simulink model "BLDC_simscape"  (R2025b)
settings: Solver=ode23t  StartTime=0.0  StopTime=10.0  RelTol=1e-3
undefined symbols (not defined in the file or in its folder): Mosfet_class, PermanentMagnetSynchrono_class
libraries: nesl_utility x26, fl_lib x22, ee_lib x10, simulink x6, eeTransforms x2, elec_conv_HighZElecRef x1, slpidlib x1
(part 2 of 2)

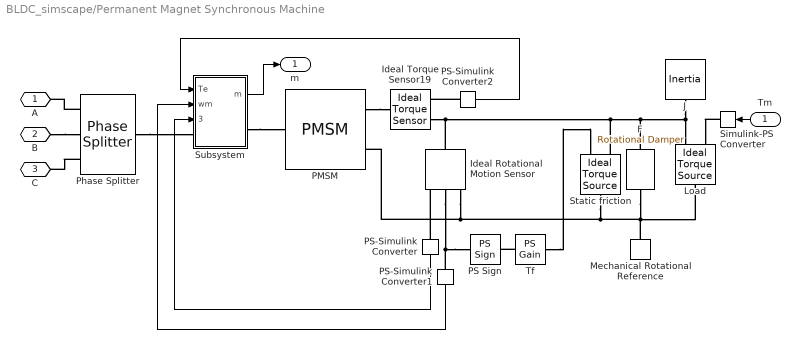
== system BLDC_simscape/Permanent Magnet Synchronous Machine ==
  Tm : Inport
  F : fl_lib/Mechanical/Rotational Elements/Rotational Damper  D=0.0004924 N*m/(rad/s)  w_specify=on  w_priority=High  w=0 rad/s  w_nominal_specify=off  w_nominal_value=1  w_nominal_unit=rad/s  t_specify=off  t_priority=None  t=0 N*m  t_nominal_specify=off  t_nominal_value=1  t_nominal_unit=N*m
  Ideal Rotational Motion Sensor : fl_lib/Mechanical/Mechanical Sensors/Ideal Rotational Motion Sensor  reference=foundation.enum.MeasurementReference.difference  acceleration_port=false  velocity_port=true  position_port=true  wrap_angle=simscape.enum.onoff.off  offset=0 deg
  Ideal Torque Sensor19 : fl_lib/Mechanical/Mechanical Sensors/Ideal Torque Sensor
  J : fl_lib/Mechanical/Rotational Elements/Inertia  inertia=0.0027 kg*m^2  num_ports=foundation.enum.numPorts2.one  w_specify=on  w_priority=High  w=0 rad/s  w_nominal_specify=off  w_nominal_value=1  w_nominal_unit=rad/s  t_specify=off  t_priority=None  t=0 N*m  t_nominal_specify=off  t_nominal_value=1  t_nominal_unit=N*m
  Load : fl_lib/Mechanical/Mechanical Sources/Ideal Torque Source
  Mechanical Rotational Reference : fl_lib/Mechanical/Rotational Elements/Mechanical Rotational Reference
  PMSM : ee_lib/Electromechanical/Permanent Magnet/PMSM  port_option=ee.enum.threePhasePort.composite  winding_type=ee.enum.statorconnection.wye  machine_param=ee.enum.pmsm.parameterization.constant  nPolePairs=4  pmflux_param=1  pm_flux_linkage=PermanentMagnetSynchrono_class('Torque Tm',[0.0027 0.0004924 4 0],4,'Flux linkage established by magnets (V.s)',0.1194,86.6271,0.7164,'90 degrees behind phase A axis (modified Park)',[0 0 0 0],'Sinusoidal',120,'3',[0 0 0 0 0 0]).objParamMappingDerived.NewDerivedParam.pm_flux_linkage Wb  torque_constant=0.18 N*m/A  back_emf_constant=0.18 V/(rad/s)  stator_param=1  Ld=0.000395 H  Lq=0.000395 H  idVec=[-200, 0, 200] A  iqVec=[-200, 0, 200] A  LdMatrix=0.0002 * ones(3, 3) H  LqMatrix=0.0002 * ones(3, 3) H  PmMatrix=0.1 * ones(3, 3) Wb  ktMatrix=0.18 * ones(3, 3) N*m/A  keMatrix=0.18 * ones(3, 3) V/(rad/s)  L0=1e-09 H  Ls=0.0002 H  Lm=-0.00002 H  Ms=0.00002 H  Rs=0.7 Ohm  zero_sequence=0  axes_param=1  loss_param=ee.enum.ironloss.none  losses_oc=[0, 0, 0] W  losses_sc=[0, 0, 0] W  f_losses=60 Hz  Isc_losses=95 A  J=0 kg*m^2  lam=0 N*m/(rad/s)  i_d_specify=on  i_d_priority=High  i_d=PermanentMagnetSynchrono_class('Torque Tm',[0.0027 0.0004924 4 0],4,'Flux linkage established by magnets (V.s)',0.1194,86.6271,0.7164,'90 degrees behind phase A axis (modified Park)',[0 0 0 0],'Sinusoidal',120,'3',[0 0 0 0 0 0]).objParamMappingDerived.NewDerivedParam.i_d A  i_d_nominal_specify=off  i_d_nominal_value=1  i_d_nominal_unit=A  i_q_specify=on  i_q_priority=High  i_q=PermanentMagnetSynchrono_class('Torque Tm',[0.0027 0.0004924 4 0],4,'Flux linkage established by magnets (V.s)',0.1194,86.6271,0.7164,'90 degrees behind phase A axis (modified Park)',[0 0 0 0],'Sinusoidal',120,'3',[0 0 0 0 0 0]).objParamMappingDerived.NewDerivedParam.i_q A  i_q_nominal_specify=off  i_q_nominal_value=1  i_q_nominal_unit=A  torque_specify=off  torque_priority=None  torque=0 N*m  torque_nominal_specify=off  torque_nominal_value=1  torque_nominal_unit=N*m  angular_velocity_specify=on  angular_velocity_priority=High  angular_velocity=0 rad/s  angular_velocity_nominal_specify=off  angular_velocity_nominal_value=1  angular_velocity_nominal_unit=rpm  angular_position_specify=on  angular_position_priority=High  angular_position=0 deg  angular_position_nominal_specify=off  angular_position_nominal_value=1  angular_position_nominal_unit=deg  alpha=3.93e-3 1/K  alpha_flux=-0.001 1/K  Tmeas=298.15 K  stator_thermal_mass=100 J/K  rotor_thermal_mass=200 J/K  Rm_percent_rotor=90  Rd_percent_rotor=30  temperatureA_specify=off  temperatureA_priority=High  temperatureA=25 degC  temperatureA_nominal_specify=off  temperatureA_nominal_value=1  temperatureA_nominal_unit=degC  temperatureB_specify=off  temperatureB_priority=High  temperatureB=25 degC  temperatureB_nominal_specify=off  temperatureB_nominal_value=1  temperatureB_nominal_unit=degC  temperatureC_specify=off  temperatureC_priority=High  temperatureC=25 degC  temperatureC_nominal_specify=off  temperatureC_nominal_value=1  temperatureC_nominal_unit=degC  temperatureR_specify=off  temperatureR_priority=High  temperatureR=25 degC  temperatureR_nominal_specify=off  temperatureR_nominal_value=1  temperatureR_nominal_unit=degC
      settings: InternalSimscapePortConfiguration="{\"Bottom\":[],\"Left\":[{\"id\":\"N\",\"label\":\"~\",\"type\":\"foundation.electrical.three_phase\"}],\"Right\":[{\"id\":\"R\",\"label\":\"R\",\"type\":\"foundation.mechanical.rotational.rotational\"},{\"id\":\"C\",\"label\":\"C\",\"type\":\"foundation.mechanical.rotational.rotational\"}],\"Top\":[]}"
  PS Sign : fl_lib/Physical Signals/Nonlinear Operators/PS Sign
      settings: InternalSimscapePortConfiguration="{\"Bottom\":[],\"Left\":[{\"id\":\"I\",\"label\":\"\",\"type\":\"input\"}],\"Right\":[{\"id\":\"O\",\"label\":\"\",\"type\":\"output\"}],\"Top\":[]}"
  PS-Simulink Converter : nesl_utility/PS-Simulink Converter  PhysicalDomain=network_engine_domain  SubClassName=ps_output  LeftPortType=input  RightPortType=output  PseudoPeriodic=off  Frequencies=[]  VectorFormat=1-D array  Unit=1  AffineConversion=off
  PS-Simulink Converter1 : nesl_utility/PS-Simulink Converter  PhysicalDomain=network_engine_domain  SubClassName=ps_output  LeftPortType=input  RightPortType=output  PseudoPeriodic=off  Frequencies=[]  VectorFormat=1-D array  Unit=1  AffineConversion=off
  PS-Simulink Converter2 : nesl_utility/PS-Simulink Converter  PhysicalDomain=network_engine_domain  SubClassName=ps_output  LeftPortType=input  RightPortType=output  PseudoPeriodic=off  Frequencies=[]  VectorFormat=1-D array  Unit=1  AffineConversion=off
  Phase Splitter : ee_lib/Connectors & References/Phase Splitter
  Simulink-PS Converter : nesl_utility/Simulink-PS Converter  PhysicalDomain=network_engine_domain  SubClassName=ps_input  LeftPortType=input  RightPortType=output  PseudoPeriodic=off  Frequencies=[]  NoiseDistribution=none  NoiseParameters=[]  Unit=1  AffineConversion=off  FilteringAndDerivatives=provide  SimscapeFilterOrder=1  InputFilterTimeConstant=0.001  UdotUserProvided=0
  Static friction : fl_lib/Mechanical/Mechanical Sources/Ideal Torque Source
  Subsystem : Subsystem
  Tf : fl_lib/Physical Signals/Functions/PS Gain  gain=PermanentMagnetSynchrono_class('Torque Tm',[0.0027 0.0004924 4 0],4,'Flux linkage established by magnets (V.s)',0.1194,86.6271,0.7164,'90 degrees behind phase A axis (modified Park)',[0 0 0 0],'Sinusoidal',120,'3',[0 0 0 0 0 0]).objParamMappingDerived.NewDerivedParam.Tf
  A : PMIOPort  Side=Left
  B : PMIOPort  Port=2  Side=Left
  C : PMIOPort  Port=3  Side=Left
  m : Outport  VectorParamsAs1DForOutWhenUnconnected=off
  wires:
  PS-Simulink Converter1/1 -> Subsystem/2(wm)
  PS-Simulink Converter/1 -> Subsystem/3(thetam)
  PS-Simulink Converter2/1 -> Subsystem/1(Te)
  Subsystem/1(m) -> m/1
  Tm/1 -> Simulink-PS Converter/1
  connections:
  PS-Simulink Converter2/LConn1 -- Ideal Torque Sensor19/RConn2
  Phase Splitter/LConn1 -- Subsystem/LConn1
  Subsystem/RConn1 -- PMSM/LConn1
  PS-Simulink Converter/LConn1 -- Ideal Rotational Motion Sensor/RConn3
  Tf/RConn1 -- Static friction/RConn1
  PS Sign/LConn1 -- PS-Simulink Converter1/LConn1 -- Ideal Rotational Motion Sensor/RConn2
  Tf/LConn1 -- PS Sign/RConn1
  PMSM/RConn1 -- Ideal Torque Sensor19/LConn1
  Ideal Torque Sensor19/RConn1 -- Static friction/RConn2 -- F/LConn1 -- Load/RConn2 -- J/LConn1 -- Ideal Rotational Motion Sensor/LConn1
  Phase Splitter/RConn3 -- C/RConn1
  Phase Splitter/RConn1 -- A/RConn1
  B/RConn1 -- Phase Splitter/RConn2
  Simulink-PS Converter/RConn1 -- Load/RConn1
  Load/LConn1 -- F/RConn1 -- Static friction/LConn1 -- PMSM/RConn2 -- Ideal Rotational Motion Sensor/RConn1 -- Mechanical Rotational Reference/LConn1

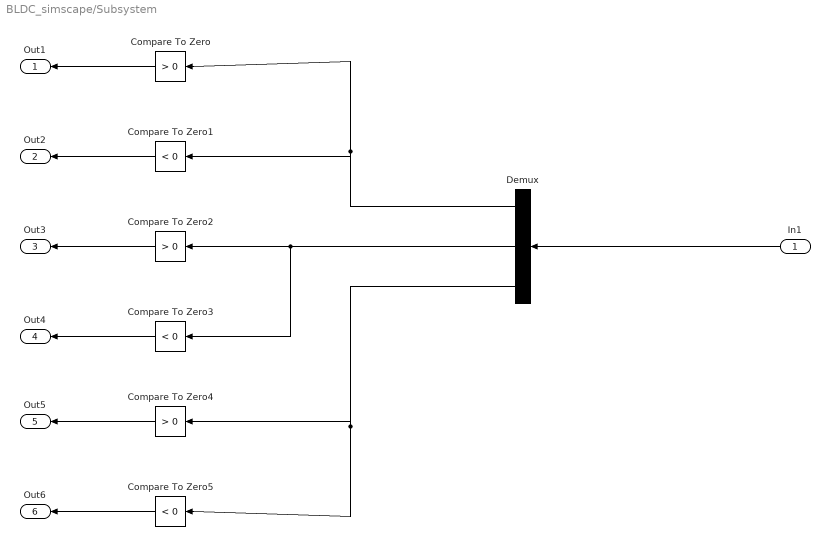
== system BLDC_simscape/Subsystem ==
  In1 : Inport
  Compare To Zero : simulink/Logic and Bit Operations/Compare To Zero  relop=>  OutDataTypeStr=boolean
  Compare To Zero1 : simulink/Logic and Bit Operations/Compare To Zero  relop=<  OutDataTypeStr=boolean
  Compare To Zero2 : simulink/Logic and Bit Operations/Compare To Zero  relop=>  OutDataTypeStr=boolean
  Compare To Zero3 : simulink/Logic and Bit Operations/Compare To Zero  relop=<  OutDataTypeStr=boolean
  Compare To Zero4 : simulink/Logic and Bit Operations/Compare To Zero  relop=>  OutDataTypeStr=boolean
  Compare To Zero5 : simulink/Logic and Bit Operations/Compare To Zero  relop=<  OutDataTypeStr=boolean
  Demux : Demux  Outputs=3
  Out1 : Outport
  Out2 : Outport  Port=2
  Out3 : Outport  Port=3
  Out4 : Outport  Port=4
  Out5 : Outport  Port=5
  Out6 : Outport  Port=6
  wires:
  Compare To Zero/1 -> Out1/1
  Compare To Zero1/1 -> Out2/1
  Compare To Zero3/1 -> Out4/1
  Compare To Zero2/1 -> Out3/1
  Compare To Zero4/1 -> Out5/1
  Compare To Zero5/1 -> Out6/1
  Demux/1 -> Compare To Zero/1, Compare To Zero1/1
  Demux/3 -> Compare To Zero4/1, Compare To Zero5/1
  Demux/2 -> Compare To Zero3/1, Compare To Zero2/1
  In1/1 -> Demux/1

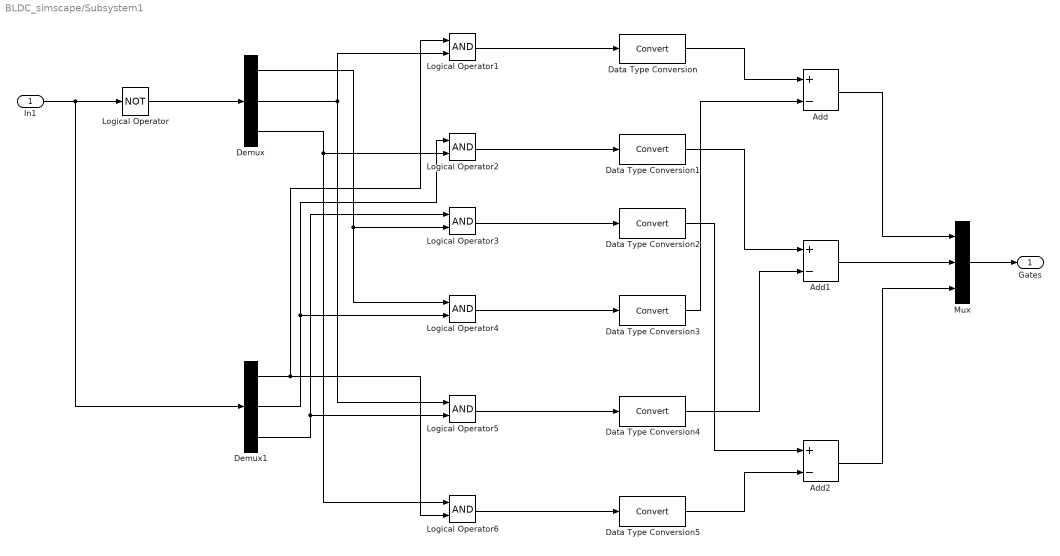
== system BLDC_simscape/Subsystem1 ==
  In1 : Inport
  Add : Sum  Inputs=+-
  Add1 : Sum  Inputs=+-
  Add2 : Sum  Inputs=+-
  Data Type Conversion{,1..5} (6 alike) : DataTypeConversion  SaturateOnIntegerOverflow=off  RndMeth=Floor
  Demux : Demux  Outputs=3
  Demux1 : Demux  Outputs=3
  Logical Operator : Logic  Operator=NOT  AllPortsSameDT=off  OutDataTypeStr=boolean
  Logical Operator{1..6} (6 alike) : Logic  AllPortsSameDT=off  OutDataTypeStr=boolean
  Mux : Mux  Inputs=3
  Gates : Outport
  wires:
  In1/1 -> Demux1/1, Logical Operator/1
  Logical Operator/1 -> Demux/1
  Logical Operator1/1 -> Data Type Conversion/1
  Data Type Conversion/1 -> Add/1
  Logical Operator2/1 -> Data Type Conversion1/1
  Logical Operator3/1 -> Data Type Conversion2/1
  Logical Operator4/1 -> Data Type Conversion3/1
  Logical Operator5/1 -> Data Type Conversion4/1
  Logical Operator6/1 -> Data Type Conversion5/1
  Data Type Conversion5/1 -> Add2/2
  Data Type Conversion1/1 -> Add1/1
  Data Type Conversion2/1 -> Add2/1
  Data Type Conversion3/1 -> Add/2
  Data Type Conversion4/1 -> Add1/2
  Mux/1 -> Gates/1
  Add/1 -> Mux/1
  Add1/1 -> Mux/2
  Add2/1 -> Mux/3
  Demux/1 -> Logical Operator3/2, Logical Operator4/1
  Demux/2 -> Logical Operator1/2, Logical Operator5/1
  Demux/3 -> Logical Operator6/1, Logical Operator2/2
  Demux1/1 -> Logical Operator6/2, Logical Operator1/1
  Demux1/2 -> Logical Operator2/1, Logical Operator4/2
  Demux1/3 -> Logical Operator5/2, Logical Operator3/1

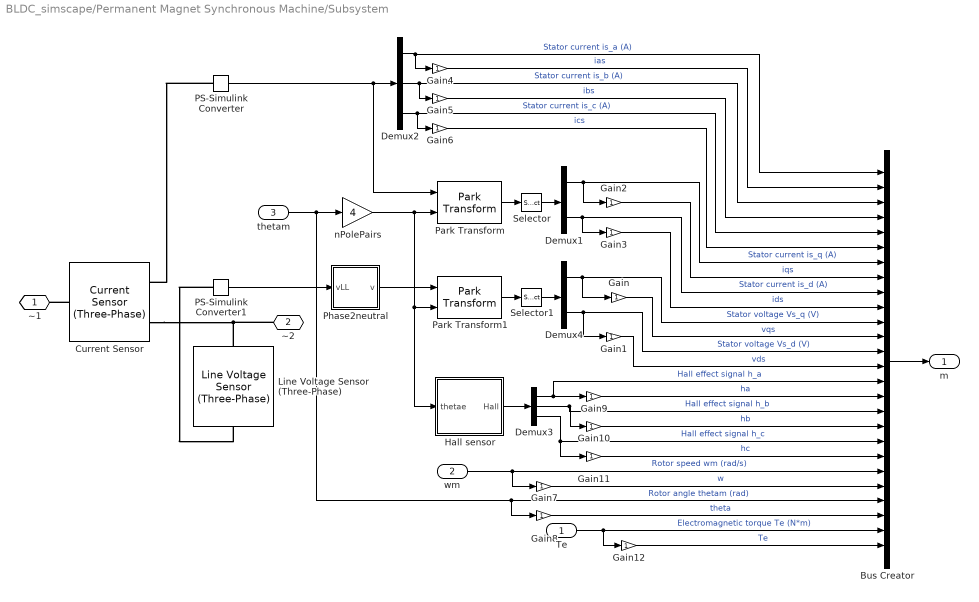
== system BLDC_simscape/Permanent Magnet Synchronous Machine/Subsystem ==
  Te : Inport
  wm : Inport  Port=2
  thetam : Inport  Port=3
  Bus Creator : BusCreator  Inputs=26
  Current Sensor : ee_lib/Sensors & Transducers/Current Sensor (Three-Phase)
  Demux1 : Demux  Outputs=2
  Demux2 : Demux  Outputs=3
  Demux3 : Demux  Outputs=3
  Demux4 : Demux  Outputs=2
  Gain{,1..12} (13 alike) : Gain
  Hall sensor : Subsystem
  Line Voltage Sensor (Three-Phase) : ee_lib/Sensors & Transducers/Line Voltage Sensor (Three-Phase)
  PS-Simulink Converter : nesl_utility/PS-Simulink Converter  PhysicalDomain=network_engine_domain  SubClassName=ps_output  LeftPortType=input  RightPortType=output  PseudoPeriodic=off  Frequencies=[]  VectorFormat=1-D array  Unit=1  AffineConversion=off
  PS-Simulink Converter1 : nesl_utility/PS-Simulink Converter  PhysicalDomain=network_engine_domain  SubClassName=ps_output  LeftPortType=input  RightPortType=output  PseudoPeriodic=off  Frequencies=[]  VectorFormat=1-D array  Unit=1  AffineConversion=off
  Park Transform : eeTransforms/Park Transform  AxisAlignment=Q-axis  PowerInvariant=off
  Park Transform1 : eeTransforms/Park Transform  AxisAlignment=Q-axis  PowerInvariant=off
  Phase2neutral : Subsystem
  Selector : Selector  InputPortWidth=3  IndexOptions=Index vector (dialog)  Indices=[2 1]  OutputSizes=1
  Selector1 : Selector  InputPortWidth=3  IndexOptions=Index vector (dialog)  Indices=[2 1]  OutputSizes=1
  nPolePairs : Gain  Gain=4
  ~1 : PMIOPort  Side=Left
  ~2 : PMIOPort  Port=2  Side=Right
  m : Outport  VectorParamsAs1DForOutWhenUnconnected=off
  wires:
  Phase2neutral/1(v) -> Park Transform1/1
  Gain8/1 -> Bus Creator/24  "theta"
  Gain7/1 -> Bus Creator/22  "w"
  Selector1/1 -> Demux4/1
  Selector/1 -> Demux1/1
  Gain11/1 -> Bus Creator/20  "hc"
  Gain10/1 -> Bus Creator/18  "hb"
  Gain9/1 -> Bus Creator/16  "ha"
  Gain1/1 -> Bus Creator/14  "vds"
  Gain/1 -> Bus Creator/12  "vqs"
  Gain3/1 -> Bus Creator/10  "ids"
  Gain2/1 -> Bus Creator/8  "iqs"
  Hall sensor/1(Hall) -> Demux3/1
  PS-Simulink Converter1/1 -> Phase2neutral/1(vLL)
  Gain6/1 -> Bus Creator/6  "ics"
  Gain5/1 -> Bus Creator/4  "ibs"
  Gain4/1 -> Bus Creator/2  "ias"
  PS-Simulink Converter/1 -> Demux2/1, Park Transform/1
  Te/1 -> Bus Creator/25, Gain12/1  "Electromagnetic torque Te (N*m)"
  Gain12/1 -> Bus Creator/26  "Te"
  Demux3/3 -> Bus Creator/19, Gain11/1  "Hall effect signal h_c"
  Demux3/2 -> Gain10/1, Bus Creator/17  "Hall effect signal h_b"
  Demux3/1 -> Gain9/1, Bus Creator/15  "Hall effect signal h_a"
  thetam/1 -> nPolePairs/1, Gain8/1, Bus Creator/23  "Rotor angle thetam (rad)"
  Bus Creator/1 -> m/1
  Demux2/3 -> Bus Creator/5, Gain6/1  "Stator current is_c (A)"
  Demux2/2 -> Gain5/1, Bus Creator/3  "Stator current is_b (A)"
  Demux2/1 -> Gain4/1, Bus Creator/1  "Stator current is_a (A)"
  Demux1/2 -> Gain3/1, Bus Creator/9  "Stator current is_d (A)"
  Park Transform/1 -> Selector/1
  Demux1/1 -> Gain2/1, Bus Creator/7  "Stator current is_q (A)"
  Demux4/2 -> Gain1/1, Bus Creator/13  "Stator voltage Vs_d (V)"
  Demux4/1 -> Gain/1, Bus Creator/11  "Stator voltage Vs_q (V)"
  Park Transform1/1 -> Selector1/1
  nPolePairs/1 -> Hall sensor/1(thetae), Park Transform1/2, Park Transform/2
  wm/1 -> Bus Creator/21, Gain7/1  "Rotor speed wm (rad/s)"
  connections:
  PS-Simulink Converter1/LConn1 -- Line Voltage Sensor (Three-Phase)/RConn1
  PS-Simulink Converter/LConn1 -- Current Sensor/RConn1
  ~2/RConn1 -- Line Voltage Sensor (Three-Phase)/LConn1 -- Current Sensor/RConn2
  Current Sensor/LConn1 -- ~1/RConn1

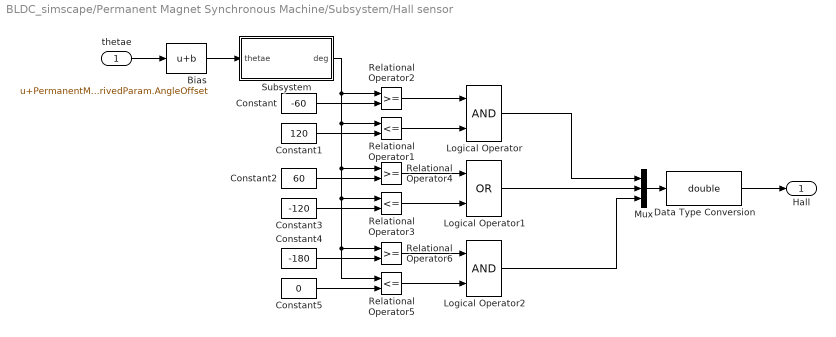
== system BLDC_simscape/Permanent Magnet Synchronous Machine/Subsystem/Hall sensor ==
  thetae : Inport
  Bias : Bias  Bias=PermanentMagnetSynchrono_class('Torque Tm',[0.0027 0.0004924 4 0],4,'Flux linkage established by magnets (V.s)',0.1194,86.6271,0.7164,'90 degrees behind phase A axis (modified Park)',[0 0 0 0],'Sinusoidal',120,'3',[0 0 0 0 0 0]).objParamMappingDerived.NewDerivedParam.AngleOffset  SaturateOnIntegerOverflow=off
  Constant : Constant  Value=-60
  Constant1 : Constant  Value=120
  Constant2 : Constant  Value=60
  Constant3 : Constant  Value=-120
  Constant4 : Constant  Value=-180
  Constant5 : Constant  Value=0
  Data Type Conversion : DataTypeConversion  OutDataTypeStr=double  SaturateOnIntegerOverflow=off  RndMeth=Floor
  Logical Operator : Logic  AllPortsSameDT=off  OutDataTypeStr=boolean
  Logical Operator1 : Logic  Operator=OR  AllPortsSameDT=off  OutDataTypeStr=boolean
  Logical Operator2 : Logic  AllPortsSameDT=off  OutDataTypeStr=boolean
  Mux : Mux  Inputs=3
  Relational Operator1 : RelationalOperator  Operator=<=
  Relational Operator2 : RelationalOperator
  Relational Operator3 : RelationalOperator  Operator=<=
  Relational Operator4 : RelationalOperator
  Relational Operator5 : RelationalOperator  Operator=<=
  Relational Operator6 : RelationalOperator
  Subsystem : Subsystem
  Hall : Outport  VectorParamsAs1DForOutWhenUnconnected=off
  wires:
  Bias/1 -> Subsystem/1(thetae)
  Data Type Conversion/1 -> Hall/1
  thetae/1 -> Bias/1
  Constant2/1 -> Relational Operator4/2
  Constant1/1 -> Relational Operator1/2
  Relational Operator4/1 -> Logical Operator1/1
  Constant/1 -> Relational Operator2/2
  Subsystem/1(deg) -> Relational Operator2/1, Relational Operator1/1, Relational Operator6/1, Relational Operator5/1, Relational Operator3/1, Relational Operator4/1
  Relational Operator1/1 -> Logical Operator/2
  Relational Operator2/1 -> Logical Operator/1
  Mux/1 -> Data Type Conversion/1
  Relational Operator3/1 -> Logical Operator1/2
  Constant5/1 -> Relational Operator5/2
  Constant4/1 -> Relational Operator6/2
  Relational Operator6/1 -> Logical Operator2/1
  Relational Operator5/1 -> Logical Operator2/2
  Logical Operator/1 -> Mux/1
  Logical Operator1/1 -> Mux/2
  Logical Operator2/1 -> Mux/3
  Constant3/1 -> Relational Operator3/2

== system BLDC_simscape/Permanent Magnet Synchronous Machine/Subsystem/Phase2neutral ==
  vLL : Inport
  Mux9 : Mux  Inputs=3
  a : Fcn  Expr=( 2*u[1] + u[2] ) / 3
  b : Fcn  Expr=( u[2] - u[1] ) / 3
  c : Fcn  Expr=( -u[1] - 2*u[2] ) / 3
  v : Outport
  wires:
  b/1 -> Mux9/2
  vLL/1 -> b/1, c/1, a/1
  c/1 -> Mux9/3
  a/1 -> Mux9/1
  Mux9/1 -> v/1

== system BLDC_simscape/Permanent Magnet Synchronous Machine/Subsystem/Hall sensor/Subsystem ==
  thetae : Inport
  Trigonometric Function : Trigonometry  Operator=sincos
  Trigonometric Function2 : Trigonometry  Operator=atan2
  rad->deg : Gain  Gain=180/pi  SaturateOnIntegerOverflow=on  OutDataTypeStr=Inherit: Same as input  ParamDataTypeStr=Inherit: Same as input
  deg : Outport  VectorParamsAs1DForOutWhenUnconnected=off
  wires:
  thetae/1 -> Trigonometric Function/1
  Trigonometric Function/2 -> Trigonometric Function2/2
  rad->deg/1 -> deg/1
  Trigonometric Function/1 -> Trigonometric Function2/1
  Trigonometric Function2/1 -> rad->deg/1
